simulink model "MPC_Boost"  (R2025a)
settings: Solver=VariableStepAuto  StartTime=0.0  StopTime=5  RelTol=1e-3
libraries: spsSeriesRLCBranchLib x4, spsVoltageMeasurementLib x2, simulink x1, spsCurrentMeasurementLib x1, spsDiodeLib x1, spsDCVoltageSourceLib x1, spsIdealSwitchLib x1, spsMosfetLib x1, slpidlib x1, sps_lib x1
settings Model: Creator=BORA  LastModifiedBy=BORA

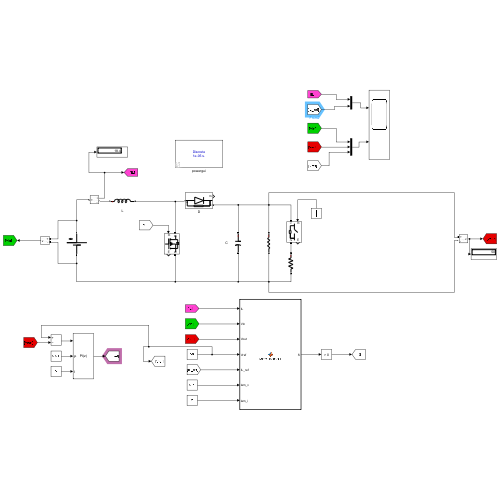
[thumbnail: Simulink's stored preview of the top-level diagram]
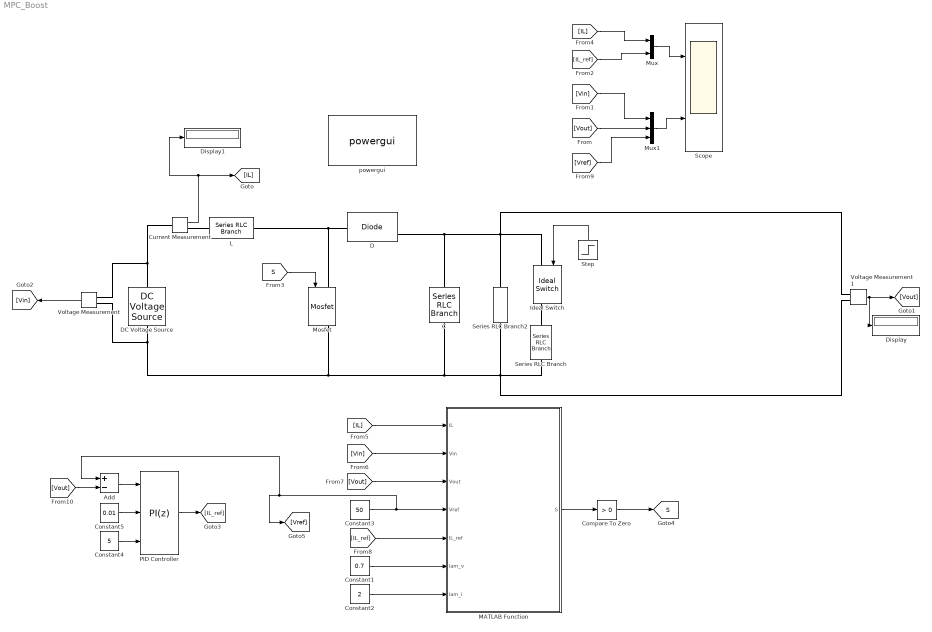
== system MPC_Boost ==
  Add : Sum  Inputs=+-
  C : spsSeriesRLCBranchLib/Series RLC Branch  LConnTagsString=__new0  RConnTagsString=__new0  BranchType=C  Resistance=1  Inductance=1e-3  SetiL0=off  InitialCurrent=0  Capacitance=37e-4  Setx0=off  InitialVoltage=0  Measurements=None
  Compare To Zero : simulink/Logic and Bit Operations/Compare To Zero  relop=>  OutDataTypeStr=boolean
  Constant1 : Constant  Value=0.7
  Constant2 : Constant  Value=2
  Constant3 : Constant  Value=50
  Constant4 : Constant  Value=5
  Constant5 : Constant  Value=0.01
  Current Measurement : spsCurrentMeasurementLib/Current Measurement  PhasorSimulation=off  OutputType=Complex  PSBequivalent=0
  D : spsDiodeLib/Diode  Ron=0.001  Lon=0  Vf=0.8  IC=0  UseSnubber=0  Rs=500  Cs=250e-9  Measurements=on
  DC Voltage Source : spsDCVoltageSourceLib/DC Voltage Source  Amplitude=30  Measurements=None
  Display : Display
  Display1 : Display
  Ideal Switch : spsIdealSwitchLib/Ideal Switch  Ron=0.001  Lon=0  IC=0  Rs=1e5  Cs=inf  Measurements=on
  L : spsSeriesRLCBranchLib/Series RLC Branch  LConnTagsString=__new0  RConnTagsString=__new0  BranchType=L  Resistance=1  Inductance=280e-4  SetiL0=off  InitialCurrent=0  Capacitance=1e-6  Setx0=off  InitialVoltage=0  Measurements=None
  MATLAB Function : MATLAB Function  TreatAsAtomicUnit=on
  Mosfet : spsMosfetLib/Mosfet  Ron=0.001  Lon=0  Rd=0.001  Vfd=0  IC=0  Rs=1e5  Cs=inf  Measurements=on
  Mux : Mux  Inputs=2
  Mux1 : Mux  Inputs=3
  PID Controller : slpidlib/PID Controller  Controller=PI  Form=Parallel  TimeDomain=Discrete-time  UseExternalTs=off  SampleTime=-1  IntegratorMethod=Forward Euler  FilterMethod=Forward Euler  ControllerParametersSource=external  P=1  I=1  UseKiTs=off  D=0  UseExternalDerivativeSource=off  N=100  UseFilter=on  TunerSelectOption=Transfer Function Based (PID Tuner App)  InitialConditionSource=internal  InitialConditionForIntegrator=0  InitialConditionForFilter=0  DifferentiatorICPrevScaledInput=0  ExternalReset=none  TrackingMode=off  Kt=1  LimitOutput=off  SatLimitsSource=internal  UpperSaturationLimit=inf  LowerSaturationLimit=-inf  LinearizeAsGain=on  AntiWindupMode=none  Kb=1  LimitIntegrator=off  UpperIntegratorSaturationLimit=inf  LowerIntegratorSaturationLimit=-inf  POutMin=[]  POutMax=[]  IOutMin=[]  IOutMax=[]  DOutMin=[]  DOutMax=[]  NOutMin=[]  NOutMax=[]  SumOutMin=[]  SumOutMax=[]  SaturationOutMin=[]  SaturationOutMax=[]  PParamMin=[]  PParamMax=[]  IParamMin=[]  IParamMax=[]  DParamMin=[]  DParamMax=[]  NParamMin=[]  NParamMax=[]  KbParamMin=[]  KbParamMax=[]  KtParamMin=[]  KtParamMax=[]  KbOutMin=[]  KbOutMax=[]  KtOutMin=[]  KtOutMax=[]  IntegratorOutMin=[]  IntegratorOutMax=[]  FilterOutMin=[]  FilterOutMax=[]  SumI1OutMin=[]  SumI1OutMax=[]  SumI2OutMin=[]  SumI2OutMax=[]  SumI3OutMin=[]  SumI3OutMax=[]  SumI4OutMin=[]  SumI4OutMax=[]  SumDOutMin=[]  SumDOutMax=[]  DifferentiatorOutMin=[]  DifferentiatorOutMax=[]  FilterDiffOutCoefMin=[]  FilterDiffOutCoefMax=[]  ReciprocalOutMin=[]  ReciprocalOutMax=[]  SumDenOutMin=[]  SumDenOutMax=[]  SumNumOutMin=[]  SumNumOutMax=[]  DivideOutMin=[]  DivideOutMax=[]  UdiffTsProdOutMin=[]  UdiffTsProdOutMax=[]  NTsProdOutMin=[]  NTsProdOutMax=[]  UintegralTsProdOutMin=[]  UintegralTsProdOutMax=[]  UngainTsProdOutMin=[]  UngainTsProdOutMax=[]  ClampingZeroOutDataTypeStr=Inherit: Inherit via back propagation  ClampingZeroOutMin=[]  ClampingZeroOutMax=[]  FilterDenConstantOutDataTypeStr=Inherit: Inherit via back propagation  FilterDenConstantOutMin=[]  FilterDenConstantOutMax=[]  PCopyOutDataTypeStr=Inherit: Inherit via back propagation  PCopyOutMin=[]  PCopyOutMax=[]  NCopyOutDataTypeStr=Inherit: Inherit via back propagation  NCopyOutMin=[]  NCopyOutMax=[]  IntegratorContinuousStateAttributes=''  IntegratorStateMustResolveToSignalObject=off  IntegratorRTWStateStorageClass=Auto  FilterContinuousStateAttributes=''  FilterStateMustResolveToSignalObject=off  FilterRTWStateStorageClass=Auto  ParallelPVariant=ExternalParameters  IdealPVariant=Disabled  IVariant=ExternalParameters  DVariant=Disabled  IntegratorVariant=Discrete  SatVariant=Disabled  AWVariant=Passthrough  PCopyVariant=Disabled  TRVariant=Disabled  FdbkBlocksVariant=Forward  IdealPFdbkVariant=Disabled  SatFdbkVariant=Disabled  DerivativeFilterVariant=Disabled  NVariant=Disabled  NCopyVariant=Disabled_SignalSpec  FilterICVariant=Disabled  IntegratorICVariant=InternalICs  ExternalResetVariant=Disabled  TRSumVariant=Passthrough  SumFdbkVariant=Disabled  SumVariant=Sum_PI  TsampFilterVariant=InternalTs  TsampNgainVariant=Passthrough  TsampIntegralVariant=Disabled_SignalSpec  ExternalSaturationOutDataTypeStr=Inherit: Same as second input  DerivativeSourceVariant=Disabled  PreIntVariant=InternalPreInt
  Scope : Scope  NumInputPorts=2
      settings: TimeSpan=10  ActiveDisplayYMinimum=-2.2944848082153837  ActiveDisplayYMaximum=20.705506007687731
  Series RLC Branch : spsSeriesRLCBranchLib/Series RLC Branch  LConnTagsString=__new0  RConnTagsString=__new0  BranchType=R  Resistance=6  Inductance=1e-3  SetiL0=off  InitialCurrent=0  Capacitance=1e-6  Setx0=off  InitialVoltage=0  Measurements=None
  Series RLC Branch2 : spsSeriesRLCBranchLib/Series RLC Branch  LConnTagsString=__new0  RConnTagsString=__new0  BranchType=R  Resistance=20  Inductance=1e-3  SetiL0=off  InitialCurrent=0  Capacitance=1e-6  Setx0=off  InitialVoltage=0  Measurements=None
  Step : Step  Time=3  SampleTime=0.0
  Voltage Measurement : spsVoltageMeasurementLib/Voltage Measurement  PhasorSimulation=off  OutputType=Complex  PSBequivalent=0
  Voltage Measurement1 : spsVoltageMeasurementLib/Voltage Measurement  PhasorSimulation=off  OutputType=Complex  PSBequivalent=0
  powergui : sps_lib/powergui  Priority=1  SimulationMode=Discrete  SampleTime=1e-05  frequency=60  Iterations=50  frequencyindice=0  Pbase=100e6  ErrMax=1e-4  UnitsV=kV  UnitsW=MW  buscounter=0  FunctionMessages=off  echomessages=off  EnableUseOfTLC=off  CurrentSourceSwitches=off  DisableSnubberDevices=off  DisableRonSwitches=off  DisableVfSwitches=off  DisplayEquations=off  AutomaticDiscreteSolvers=off  SolverType=Tustin/Backward Euler (TBE)  Interpol=off  ExternalGateDelay=off  methode=off  Ts=100  x0status=blocks  SPID=on  SwTol=0  HookPort=off  NonlinearTolerance=1e-4  nMaxIteration=100  ContinueOnMaxIteration=off  RestoreLinks=warning  ResistiveCurrentMeasurement=off  Frange=[0:2:500]  Ylog=off  Xlog=on  ShowGrid=off  save=off  variable=ZData  structure=0  ZoomFFT=off  StartTime=0.0  cycles=1  DisplayStyle=1  fundamental=60  FreqAxis=off  MaxFrequency=1000  frequencyindicesteady=1  RmsSteady=1  display=off
  tag scope: S=global
  wires:
  Current Measurement/1 -> [IL], Display1/1
  Voltage Measurement1/1 -> Display/1, [Vout]
  Voltage Measurement/1 -> [Vin]
  [IL] -> MATLAB Function/1(IL)
  [Vin] -> MATLAB Function/2(Vin)
  [Vout] -> MATLAB Function/3(Vout)
  [IL_ref] -> MATLAB Function/5(IL_ref)
  [IL_ref] -> Mux/2
  [IL] -> Mux/1
  Mux/1 -> Scope/1
  [Vin] -> Mux1/1
  [Vout] -> Mux1/2
  Mux1/1 -> Scope/2
  [S] -> Mosfet/1
  MATLAB Function/1(S) -> Compare To Zero/1
  Compare To Zero/1 -> [S]
  Constant2/1 -> MATLAB Function/7(lam_i)
  Constant1/1 -> MATLAB Function/6(lam_v)
  Constant3/1 -> Add/1, [Vref], MATLAB Function/4(Vref)
  [Vref] -> Mux1/3
  Constant5/1 -> PID Controller/2
  Constant4/1 -> PID Controller/3
  Add/1 -> PID Controller/1
  [Vout] -> Add/2
  PID Controller/1 -> [IL_ref]
  Step/1 -> Ideal Switch/1
  connections:
  DC Voltage Source/LConn1 -- Voltage Measurement/LConn2 -- Mosfet/RConn1 -- Series RLC Branch/RConn1 -- Series RLC Branch2/RConn1 -- Voltage Measurement1/LConn2 -- C/RConn1
  L/RConn1 -- Mosfet/LConn1 -- D/LConn1
  C/LConn1 -- Voltage Measurement1/LConn1 -- Series RLC Branch2/LConn1 -- Ideal Switch/LConn1 -- D/RConn1
  Current Measurement/RConn1 -- L/LConn1
  Current Measurement/LConn1 -- Voltage Measurement/LConn1 -- DC Voltage Source/RConn1
  Series RLC Branch/LConn1 -- Ideal Switch/RConn1

== matlab function MPC_Boost/MATLAB Function ==
  data: S output; IL input; Vin input; Vout input; Vref input; IL_ref input; lam_v input; lam_i input

function S = MPC_BOOST(IL, Vin, Vout, Vref, IL_ref, lam_v, lam_i)
    Ts = 10e-9;     
    L = 280e-4;       
    C = 37e-4;      
    R = 20;         
    
    persistent S_old;
    if isempty(S_old)
        S_old = 0; 
    end

    State = [1; 0];
    J_optimum = 1e6; 
    n_optimum = 1;

    for n = 1:2
        S_test = State(n);

        iL_k1 = (Ts/L) * (Vin - Vout * (1 - S_test)) + IL;
        vOut_k1 = (Ts/C) * ((1 - S_test) * IL - Vout / R) + Vout;
        J = lam_v * abs(Vref - vOut_k1) + lam_i * abs(IL_ref - iL_k1);

        if (J < J_optimum)
            n_optimum = n;
            J_optimum = J;
        end
    end
    S = State(n_optimum);
    S_old = S;
end
